simulink model "simscape_antenna_240102"  (R2022a)
settings: Solver=VariableStepAuto  StartTime=0.0  StopTime=5  FixedStep=Ts  RelTol=1e-3  AbsTol=1e-3  EnableMultiTasking=on
PreLoadFcn:
  | % Control parameters
  | Ts = 2e-6;   % Fundamental sample time
  | fsw = 2e3;   % Switching frequency (Hz)
  | fc = fsw*10; % Control loop frequency (Hz)
  | Tsc = 1/fc;  % Control loop sample time
  | 
  | % PMSM parameters
  | PM = 0.03; % Permanent magnet flux linkage
  | Ld = 2e-4;  % d-axis inductance
  | Lq = 2e-4;  % q-axis inductance
  | L0 = 2e-4;  % 0-axis inductance
  | Rs = 0.013; % Stator resistance
  | N = 6; % Number of pole pairs
  | J = 0.2; % Moment of inertia
  | 
  | % Operating and derived limits
  | Imax = 100;  % Max stator current (peak value)
  | Tmax = 1.5*N*PM*Imax; % Max lectromagnetic torque
  | fnom = 100;  % Nominal frequency (Hz)
  | rpm_nom = 60*fnom/N;      % Nominal rotor speed (rpm)
  | omegam_nom = 2*pi*fnom/N; % Nominal mechanical rotor speed
  | Pmax = omegam_nom*Tmax;     % Maximum power
StopFcn:
  | ee_addSimlogTimeStamp(bdroot)
undefined symbols (not defined in the file or in its folder): smiData, X, Y, Z
libraries: nesl_utility x21, ee_lib x20, fl_lib x20, sm_lib x15, slpidlib x6, eePwmGeneratorTwoLevel x2, spsabctodq0Lib x2, eeTransforms x2, spsdq0toabcLib x1, eePmsmCurrentController x1, eePmsmCurrentReferenceGen x1, eePmsmFieldOrientedControl x1
(part 2 of 3)

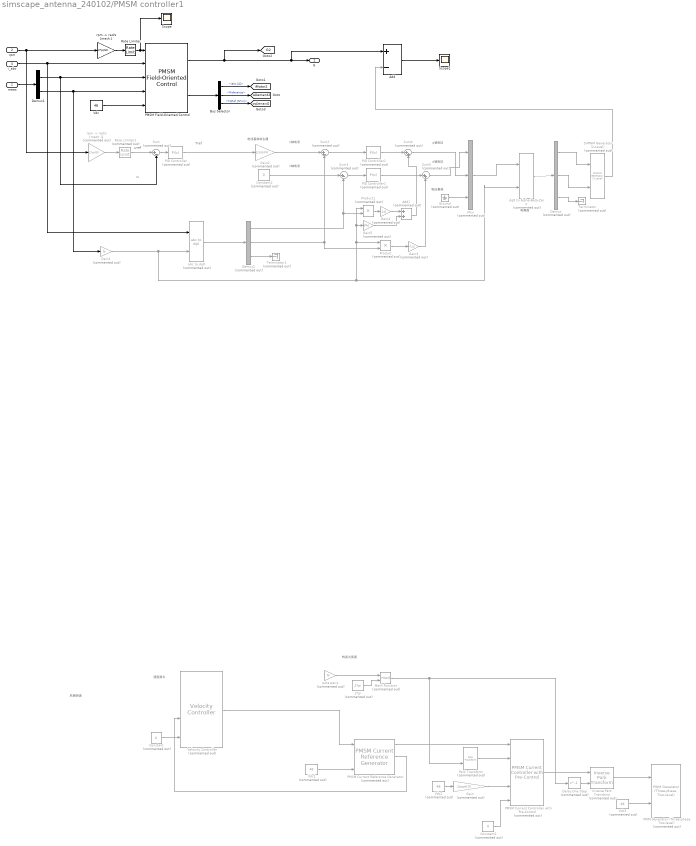
== system simscape_antenna_240102/PMSM controller1 ==
  note: 电角度
  note: 电压基准
  note: q轴电压
  note: 电流基准发生器
  note: Tref
  note: ω
  note: d轴电流
  note: q轴电流
  note: ωref
  note: 转变为弧度
  note: 速度指令
  note: 机械转速
  note: d轴电压
  meas : Inport
  rpm : Inport  Port=2
  i_abc : Inport  Port=3
  2*pi : Constant  Commented=on  Value=2*pi  SampleTime=-1
  Add : Sum  Inputs=+-
  Add1 : Sum  Commented=on
  Bus Selector : BusSelector  OutputSignals=iabc [A],Reference,TqRef [N*m]
  Constant : Constant  Commented=on  Value=0
  Constant1 : Constant  Commented=on  Value=0
  Constant2 : Constant  Commented=on  Value=0
  Delay One Step : Delay  Commented=on  DelayLength=1
  Demux : Demux  Commented=on  Outputs=3
  Demux1 : Demux  Outputs=2
  Demux2 : Demux  Commented=on  Outputs=3
  Gain : Gain  Commented=on  Gain=1/sqrt(3)
  Gain1 : Gain  Commented=on  Gain=N
  Gain2 : Gain  Commented=on  Gain=2/3/N/PM
  Gain3 : Gain  Commented=on  Gain=-Lq
  Gain4 : Gain  Commented=on  Gain=Ld
  Gain5 : Gain  Commented=on  Gain=PM
  Ground : Ground  Commented=on
  Inverse Park Transform : eeTransforms/Inverse Park Transform  Commented=on  AxisAlignment=Q-axis  PowerInvariant=off
  Math Function : Math  Commented=on  Operator=mod  SignedPower=on
  Mux : Mux  Commented=on  Inputs=3
  PID Controller : slpidlib/PID Controller  Commented=on  Controller=PI  Form=Parallel  TimeDomain=Discrete-time  UseExternalTs=off  SampleTime=-1  IntegratorMethod=Forward Euler  FilterMethod=Forward Euler  ControllerParametersSource=internal  P=60  I=6000  UseKiTs=off  D=0  N=100  UseFilter=on  TunerSelectOption=Transfer Function Based (PID Tuner App)  InitialConditionSource=internal  InitialConditionForIntegrator=0  InitialConditionForFilter=0  DifferentiatorICPrevScaledInput=0  ExternalReset=none  TrackingMode=off  Kt=1  LimitOutput=off  SatLimitsSource=internal  UpperSaturationLimit=inf  LowerSaturationLimit=-inf  LinearizeAsGain=on  AntiWindupMode=none  Kb=1  POutMin=[]  POutMax=[]  IOutMin=[]  IOutMax=[]  DOutMin=[]  DOutMax=[]  NOutMin=[]  NOutMax=[]  SumOutMin=[]  SumOutMax=[]  SaturationOutMin=[]  SaturationOutMax=[]  PParamMin=[]  PParamMax=[]  IParamMin=[]  IParamMax=[]  DParamMin=[]  DParamMax=[]  NParamMin=[]  NParamMax=[]  KbParamMin=[]  KbParamMax=[]  KtParamMin=[]  KtParamMax=[]  KbOutMin=[]  KbOutMax=[]  KtOutMin=[]  KtOutMax=[]  IntegratorOutMin=[]  IntegratorOutMax=[]  FilterOutMin=[]  FilterOutMax=[]  SumI1OutMin=[]  SumI1OutMax=[]  SumI2OutMin=[]  SumI2OutMax=[]  SumI3OutMin=[]  SumI3OutMax=[]  SumI4OutMin=[]  SumI4OutMax=[]  SumDOutMin=[]  SumDOutMax=[]  DifferentiatorOutMin=[]  DifferentiatorOutMax=[]  FilterDiffOutCoefMin=[]  FilterDiffOutCoefMax=[]  ReciprocalOutMin=[]  ReciprocalOutMax=[]  SumDenOutMin=[]  SumDenOutMax=[]  SumNumOutMin=[]  SumNumOutMax=[]  DivideOutMin=[]  DivideOutMax=[]  UdiffTsProdOutMin=[]  UdiffTsProdOutMax=[]  NTsProdOutMin=[]  NTsProdOutMax=[]  UintegralTsProdOutMin=[]  UintegralTsProdOutMax=[]  UngainTsProdOutMin=[]  UngainTsProdOutMax=[]  IntegratorContinuousStateAttributes=''  IntegratorStateMustResolveToSignalObject=off  IntegratorRTWStateStorageClass=Auto  FilterContinuousStateAttributes=''  FilterStateMustResolveToSignalObject=off  FilterRTWStateStorageClass=Auto  ParallelPVariant=InternalParameters  IdealPVariant=Disabled  IVariant=InternalParameters  DVariant=Disabled  IntegratorVariant=Discrete  SatVariant=Disabled  AWVariant=Passthrough  PCopyVariant=Disabled  TRVariant=Disabled  FdbkBlocksVariant=Forward  IdealPFdbkVariant=Disabled  SatFdbkVariant=Disabled  DerivativeFilterVariant=Disabled  NVariant=Disabled  NCopyVariant=Disabled_SignalSpec  FilterICVariant=Disabled  IntegratorICVariant=InternalICs  ExternalResetVariant=Disabled  TRSumVariant=Passthrough  SumFdbkVariant=Disabled  SumVariant=Sum_PI  TsampFilterVariant=InternalTs  TsampNgainVariant=Passthrough  TsampIntegralVariant=Passthrough  ExternalSaturationOutDataTypeStr=Inherit: Same as second input  aMode=0
  PID Controller1 : slpidlib/PID Controller  Commented=on  Controller=PI  Form=Parallel  TimeDomain=Discrete-time  UseExternalTs=off  SampleTime=-1  IntegratorMethod=Forward Euler  FilterMethod=Forward Euler  ControllerParametersSource=internal  P=0.1  I=10  UseKiTs=off  D=0  N=100  UseFilter=on  TunerSelectOption=Transfer Function Based (PID Tuner App)  InitialConditionSource=internal  InitialConditionForIntegrator=0  InitialConditionForFilter=0  DifferentiatorICPrevScaledInput=0  ExternalReset=none  TrackingMode=off  Kt=1  LimitOutput=off  SatLimitsSource=internal  UpperSaturationLimit=inf  LowerSaturationLimit=-inf  LinearizeAsGain=on  AntiWindupMode=none  Kb=1  POutMin=[]  POutMax=[]  IOutMin=[]  IOutMax=[]  DOutMin=[]  DOutMax=[]  NOutMin=[]  NOutMax=[]  SumOutMin=[]  SumOutMax=[]  SaturationOutMin=[]  SaturationOutMax=[]  PParamMin=[]  PParamMax=[]  IParamMin=[]  IParamMax=[]  DParamMin=[]  DParamMax=[]  NParamMin=[]  NParamMax=[]  KbParamMin=[]  KbParamMax=[]  KtParamMin=[]  KtParamMax=[]  KbOutMin=[]  KbOutMax=[]  KtOutMin=[]  KtOutMax=[]  IntegratorOutMin=[]  IntegratorOutMax=[]  FilterOutMin=[]  FilterOutMax=[]  SumI1OutMin=[]  SumI1OutMax=[]  SumI2OutMin=[]  SumI2OutMax=[]  SumI3OutMin=[]  SumI3OutMax=[]  SumI4OutMin=[]  SumI4OutMax=[]  SumDOutMin=[]  SumDOutMax=[]  DifferentiatorOutMin=[]  DifferentiatorOutMax=[]  FilterDiffOutCoefMin=[]  FilterDiffOutCoefMax=[]  ReciprocalOutMin=[]  ReciprocalOutMax=[]  SumDenOutMin=[]  SumDenOutMax=[]  SumNumOutMin=[]  SumNumOutMax=[]  DivideOutMin=[]  DivideOutMax=[]  UdiffTsProdOutMin=[]  UdiffTsProdOutMax=[]  NTsProdOutMin=[]  NTsProdOutMax=[]  UintegralTsProdOutMin=[]  UintegralTsProdOutMax=[]  UngainTsProdOutMin=[]  UngainTsProdOutMax=[]  IntegratorContinuousStateAttributes=''  IntegratorStateMustResolveToSignalObject=off  IntegratorRTWStateStorageClass=Auto  FilterContinuousStateAttributes=''  FilterStateMustResolveToSignalObject=off  FilterRTWStateStorageClass=Auto  ParallelPVariant=InternalParameters  IdealPVariant=Disabled  IVariant=InternalParameters  DVariant=Disabled  IntegratorVariant=Discrete  SatVariant=Disabled  AWVariant=Passthrough  PCopyVariant=Disabled  TRVariant=Disabled  FdbkBlocksVariant=Forward  IdealPFdbkVariant=Disabled  SatFdbkVariant=Disabled  DerivativeFilterVariant=Disabled  NVariant=Disabled  NCopyVariant=Disabled_SignalSpec  FilterICVariant=Disabled  IntegratorICVariant=InternalICs  ExternalResetVariant=Disabled  TRSumVariant=Passthrough  SumFdbkVariant=Disabled  SumVariant=Sum_PI  TsampFilterVariant=InternalTs  TsampNgainVariant=Passthrough  TsampIntegralVariant=Passthrough  ExternalSaturationOutDataTypeStr=Inherit: Same as second input  aMode=0
  PID Controller2 : slpidlib/PID Controller  Commented=on  Controller=PI  Form=Parallel  TimeDomain=Discrete-time  UseExternalTs=off  SampleTime=-1  IntegratorMethod=Forward Euler  FilterMethod=Forward Euler  ControllerParametersSource=internal  P=0.1  I=10  UseKiTs=off  D=0  N=100  UseFilter=on  TunerSelectOption=Transfer Function Based (PID Tuner App)  InitialConditionSource=internal  InitialConditionForIntegrator=0  InitialConditionForFilter=0  DifferentiatorICPrevScaledInput=0  ExternalReset=none  TrackingMode=off  Kt=1  LimitOutput=off  SatLimitsSource=internal  UpperSaturationLimit=inf  LowerSaturationLimit=-inf  LinearizeAsGain=on  AntiWindupMode=none  Kb=1  POutMin=[]  POutMax=[]  IOutMin=[]  IOutMax=[]  DOutMin=[]  DOutMax=[]  NOutMin=[]  NOutMax=[]  SumOutMin=[]  SumOutMax=[]  SaturationOutMin=[]  SaturationOutMax=[]  PParamMin=[]  PParamMax=[]  IParamMin=[]  IParamMax=[]  DParamMin=[]  DParamMax=[]  NParamMin=[]  NParamMax=[]  KbParamMin=[]  KbParamMax=[]  KtParamMin=[]  KtParamMax=[]  KbOutMin=[]  KbOutMax=[]  KtOutMin=[]  KtOutMax=[]  IntegratorOutMin=[]  IntegratorOutMax=[]  FilterOutMin=[]  FilterOutMax=[]  SumI1OutMin=[]  SumI1OutMax=[]  SumI2OutMin=[]  SumI2OutMax=[]  SumI3OutMin=[]  SumI3OutMax=[]  SumI4OutMin=[]  SumI4OutMax=[]  SumDOutMin=[]  SumDOutMax=[]  DifferentiatorOutMin=[]  DifferentiatorOutMax=[]  FilterDiffOutCoefMin=[]  FilterDiffOutCoefMax=[]  ReciprocalOutMin=[]  ReciprocalOutMax=[]  SumDenOutMin=[]  SumDenOutMax=[]  SumNumOutMin=[]  SumNumOutMax=[]  DivideOutMin=[]  DivideOutMax=[]  UdiffTsProdOutMin=[]  UdiffTsProdOutMax=[]  NTsProdOutMin=[]  NTsProdOutMax=[]  UintegralTsProdOutMin=[]  UintegralTsProdOutMax=[]  UngainTsProdOutMin=[]  UngainTsProdOutMax=[]  IntegratorContinuousStateAttributes=''  IntegratorStateMustResolveToSignalObject=off  IntegratorRTWStateStorageClass=Auto  FilterContinuousStateAttributes=''  FilterStateMustResolveToSignalObject=off  FilterRTWStateStorageClass=Auto  ParallelPVariant=InternalParameters  IdealPVariant=Disabled  IVariant=InternalParameters  DVariant=Disabled  IntegratorVariant=Discrete  SatVariant=Disabled  AWVariant=Passthrough  PCopyVariant=Disabled  TRVariant=Disabled  FdbkBlocksVariant=Forward  IdealPFdbkVariant=Disabled  SatFdbkVariant=Disabled  DerivativeFilterVariant=Disabled  NVariant=Disabled  NCopyVariant=Disabled_SignalSpec  FilterICVariant=Disabled  IntegratorICVariant=InternalICs  ExternalResetVariant=Disabled  TRSumVariant=Passthrough  SumFdbkVariant=Disabled  SumVariant=Sum_PI  TsampFilterVariant=InternalTs  TsampNgainVariant=Passthrough  TsampIntegralVariant=Passthrough  ExternalSaturationOutDataTypeStr=Inherit: Same as second input  aMode=0
  PMSM Current Controller with Pre-Control : eePmsmCurrentController/PMSM Current Controller with Pre-Control  Commented=on  Kp_id=0.1  Ki_id=10  Kaw_id=1000  Kp_iq=0.1  Ki_iq=10  Kaw_iq=1000  Ts=-1  Tsd=0.001  AxisPrio=Q-axis  ActZC=off  ActFF=on  idVect=[-200, 0, 200]  iqVect=[-200, 0, 200]  LdMatrix=0.0002 * ones(3, 3)  LqMatrix=0.0002 * ones(3, 3)  psimMatrix=0.04 * ones(3, 3)
      settings: SourceProductBaseCode=PS
  PMSM Current Reference Generator : eePmsmCurrentReferenceGen/PMSM Current Reference Generator  Commented=on  Vnom=10  Pmax=Pmax  Tmax=Tmax*1.5  Ts=2e-6  RefType=Zero d-axis control  rpmVec=[0, 3000]  TqVec=[-100, 0, 100]  VdcVec=[300, 350]  PWMMode=SVM: space vector modulation  ModFactor=1  idMatrix=zeros(2,3,2)  iqMatrix=zeros(2,3,2)  p=8  psim=0.04  Ld=0.00024  Lq=0.00029  Rs=0.01  RefExpEnable=0
      settings: SourceProductBaseCode=PS
  PMSM Field-Oriented Control : eePmsmFieldOrientedControl/PMSM Field-Oriented Control  winding_type=Wye-wound  CtrlMode=Velocity control  Vnom=48  Pmax=Pmax  Tmax=Tmax*1.5  p=N  Vdc_on=10  Ts=Ts  Tsc=Tsc  CtrlType=PI control  Kp_w=60  Ki_w=300*2  Kv_w=1  Kaw_w=1000  RefType=Zero d-axis control  rpmVec=[0, 3000]  TqVec=[-100, 0, 100]  VdcVec=[300, 350]  PWMMode=SPWM: sinusoidal PWM  ModFactor=1  idMatrix=zeros(2,3,2)  iqMatrix=zeros(2,3,2)  psim=PM  Ld=0.00024  Lq=0.00029  Rs=0.01  AxisAlignment=Q-axis  Kp_id=0.1  Ki_id=10  Kaw_id=1000  Kp_iq=0.1  Ki_iq=10  Kaw_iq=1000  AxisPrio=Q-axis  ActZC=off  ActFF=on  ParamTypeFF=Constant parameters  LdFF=Ld  LqFF=Lq  psimFF=PM  idVect=[-200, 0, 200]  iqVect=[-200, 0, 200]  LdMatrix=0.0002 * ones(3, 3)  LqMatrix=0.0002 * ones(3, 3)  psimMatrix=0.04 * ones(3, 3)  CPWMMode=SPWM: sinusoidal PWM  fsw=fsw
      settings: SourceProductBaseCode=PS
  "PWM Generator (Three-phase, Two-level)" : eePwmGeneratorTwoLevel/PWM Generator (Three-phase, Two-level)  Commented=on  PWMMode=Continuous PWM (CPWM)  CPWMMode=SPWM: sinusoidal PWM  DPWMMode=60 DPWM: 60 degree discontinuous PWM  fsw=1e3  Ts=2e-6
      settings: SourceProductBaseCode=PS
  Park Transform : eeTransforms/Park Transform  Commented=on  AxisAlignment=Q-axis  PowerInvariant=off
  Product : Product  Commented=on
  Product1 : Product  Commented=on
  Rate Limiter : RateLimiter  RisingSlewLimit=Tmax/J  FallingSlewLimit=-Tmax/J  SampleTimeMode=inherited
  Rate Limiter1 : RateLimiter  Commented=on  RisingSlewLimit=Tmax/J  FallingSlewLimit=-Tmax/J  SampleTimeMode=inherited
  SVPWM Generator (2-Level) : spsSVPWMGenerator2LevelLib/SVPWM Generator (2-Level)  Commented=on  InputType=alpha-beta components  SwitchingPattern=Pattern #1  Fc=2000  ParUref=[0.8 -30 50]  Ts=0
      settings: SourceProductBaseCode=PS
  Scope : Scope
  Scope1 : Scope
  Sum : Sum  Commented=on  Inputs=|+-
  Sum2 : Sum  Commented=on  Inputs=|+-
  Sum3 : Sum  Commented=on  Inputs=|+-
  Sum4 : Sum  Commented=on  Inputs=|++
  Sum5 : Sum  Commented=on  Inputs=|++
  Terminator : Terminator  Commented=on
  Terminator1 : Terminator  Commented=on
  Vdc : Constant  Value=48  SampleTime=Tsc
  Vdc1 : Constant  Commented=on  Value=48  SampleTime=Tsc
  Vdc2 : Constant  Commented=on  Value=48  SampleTime=Tsc
  Vdc3 : Constant  Commented=on  Value=48  SampleTime=Tsc
  Velocity Controller : eeVelocityController/Velocity Controller  Commented=on  CtrlType=PI control  Kp_w=60  Ki_w=300*2  Kv_w=1  Kaw_w=1000  Ts=2e-6  Tsd=0.001  ActZC=off
      settings: SourceProductBaseCode=PS
  abc to dq0 : spsabctodq0Lib/abc to dq0  Commented=on  Alignment=90 degrees behind phase A axis
  dq0 to Alpha-Beta-Zero : spsdq0toAlphaBetaZeroLib/dq0 to Alpha-Beta-Zero  Commented=on  Alignment=90 degrees behind phase A axis
      settings: SourceProductBaseCode=PS
  "pole pairs " : Gain  Commented=on  Gain=N
  "rpm -> rad/s [mech.]" : Gain  Gain=2*pi/60
  "rpm -> rad/s [mech.]1" : Gain  Commented=on  Gain=2*pi/60
  G : Outport  VectorParamsAs1DForOutWhenUnconnected=off
  tag scope: G2=global, iMotor2=global, trqDemand2=global, wDemand2=global
  wires:
  "rpm -> rad/s [mech.]"/1 -> Rate Limiter/1
  Rate Limiter/1 -> Scope/1, PMSM Field-Oriented Control/1
  rpm/1 -> "rpm -> rad/s [mech.]1"/1, "rpm -> rad/s [mech.]"/1
  Bus Selector/3 -> [trqDemand2]  "<TqRef [N*m]>"
  Bus Selector/2 -> [wDemand2]  "<Reference>"
  Bus Selector/1 -> [iMotor2]  "<iabc [A]>"
  meas/1 -> Demux1/1
  i_abc/1 -> abc to dq0/1, PMSM Field-Oriented Control/2
  PMSM Field-Oriented Control/2 -> Bus Selector/1
  Vdc/1 -> PMSM Field-Oriented Control/5
  PMSM Field-Oriented Control/1 -> G/1, Add/1, [G2]
  "rpm -> rad/s [mech.]1"/1 -> Rate Limiter1/1
  Rate Limiter1/1 -> Sum/1
  Sum/1 -> PID Controller/1
  Velocity Controller/1 -> PMSM Current Reference Generator/1
  PMSM Current Reference Generator/1 -> PMSM Current Controller with Pre-Control/1
  PMSM Current Controller with Pre-Control/1 -> Inverse Park Transform/1
  Inverse Park Transform/1 -> "PWM Generator (Three-phase, Two-level)"/1
  Constant/1 -> Velocity Controller/4
  PMSM Current Reference Generator/2 -> Velocity Controller/3
  Vdc1/1 -> PMSM Current Reference Generator/3
  Park Transform/1 -> PMSM Current Controller with Pre-Control/2
  Vdc2/1 -> Gain/1
  Gain/1 -> PMSM Current Controller with Pre-Control/4
  Constant1/1 -> PMSM Current Controller with Pre-Control/5
  Vdc3/1 -> "PWM Generator (Three-phase, Two-level)"/2
  2*pi/1 -> Math Function/2
  "pole pairs "/1 -> Math Function/1
  Demux1/2 -> Gain1/1, PMSM Field-Oriented Control/4
  Math Function/1 -> Delay One Step/1, Park Transform/2
  Add/1 -> Scope1/1
  Delay One Step/1 -> Inverse Park Transform/2
  Demux1/1 -> PMSM Field-Oriented Control/3, Sum/2
  PID Controller/1 -> Gain2/1
  Gain2/1 -> Sum2/1
  Sum2/1 -> PID Controller1/1
  Constant2/1 -> Sum3/1
  Demux2/2 -> Product/2, Sum2/2
  Demux2/1 -> Product1/2, Sum3/2
  Sum3/1 -> PID Controller2/1
  PID Controller1/1 -> Sum4/1
  PID Controller2/1 -> Sum5/1
  Sum4/1 -> Mux/2
  Sum5/1 -> Mux/1
  Ground/1 -> Mux/3
  Mux/1 -> dq0 to Alpha-Beta-Zero/1
  dq0 to Alpha-Beta-Zero/1 -> Demux/1
  Demux/1 -> SVPWM Generator (2-Level)/1
  Demux/2 -> SVPWM Generator (2-Level)/2
  Demux/3 -> Terminator/1
  SVPWM Generator (2-Level)/1 -> Add/2
  abc to dq0/1 -> Demux2/1
  Demux2/3 -> Terminator1/1
  Gain1/1 -> Gain5/1, Product1/1, Product/1, dq0 to Alpha-Beta-Zero/2, abc to dq0/2
  Gain3/1 -> Sum5/2
  Product/1 -> Gain3/1
  Product1/1 -> Gain4/1
  Gain4/1 -> Add1/1
  Gain5/1 -> Add1/2
  Add1/1 -> Sum4/2

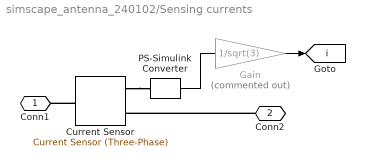
== system simscape_antenna_240102/Sensing currents ==
  Current Sensor : ee_lib/Sensors & Transducers/Current Sensor (Three-Phase)
  Gain : Gain  Commented=on  Gain=1/sqrt(3)
  PS-Simulink Converter : nesl_utility/PS-Simulink Converter  PhysicalDomain=network_engine_domain  SubClassName=ps_output  LeftPortType=input  RightPortType=output  PseudoPeriodic=off  Frequencies=[]  VectorFormat=1-D array  Unit=A  AffineConversion=off
      settings: SourceProductBaseCode=SS,PW,VE
  Conn1 : PMIOPort  Side=Left
  Conn2 : PMIOPort  Port=2  Side=Right
  tag scope: i=global
  wires:
  PS-Simulink Converter/1 -> [i]
  connections:
  Current Sensor/RConn1 -- PS-Simulink Converter/LConn1
  Conn2/RConn1 -- Current Sensor/RConn2
  Current Sensor/LConn1 -- Conn1/RConn1

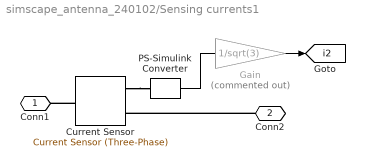
== system simscape_antenna_240102/Sensing currents1 ==
  Current Sensor : ee_lib/Sensors & Transducers/Current Sensor (Three-Phase)
  Gain : Gain  Commented=on  Gain=1/sqrt(3)
  PS-Simulink Converter : nesl_utility/PS-Simulink Converter  PhysicalDomain=network_engine_domain  SubClassName=ps_output  LeftPortType=input  RightPortType=output  PseudoPeriodic=off  Frequencies=[]  VectorFormat=1-D array  Unit=A  AffineConversion=off
      settings: SourceProductBaseCode=SS,PW,VE
  Conn1 : PMIOPort  Side=Left
  Conn2 : PMIOPort  Port=2  Side=Right
  tag scope: i2=global
  wires:
  PS-Simulink Converter/1 -> [i2]
  connections:
  Current Sensor/LConn1 -- Conn1/RConn1
  Conn2/RConn1 -- Current Sensor/RConn2
  Current Sensor/RConn1 -- PS-Simulink Converter/LConn1

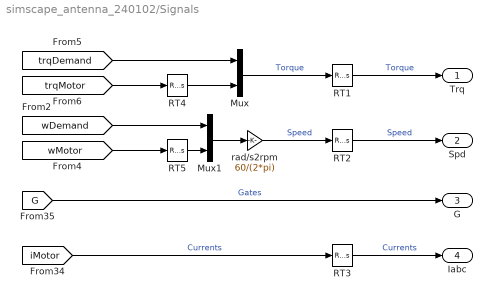
== system simscape_antenna_240102/Signals  ==
  Mux : Mux  Inputs=2
  Mux1 : Mux  Inputs=2
  RT1 : RateTransition  OutPortSampleTime=Ts
  RT2 : RateTransition  OutPortSampleTime=Ts
  RT3 : RateTransition  OutPortSampleTime=Ts
  RT4 : RateTransition  OutPortSampleTime=Tsc
  RT5 : RateTransition  OutPortSampleTime=Tsc
  rad/s2rpm : Gain  Gain=60/(2*pi)
  Trq : Outport  VectorParamsAs1DForOutWhenUnconnected=off
  Spd : Outport  Port=2  VectorParamsAs1DForOutWhenUnconnected=off
  G : Outport  Port=3  VectorParamsAs1DForOutWhenUnconnected=off
  Iabc : Outport  Port=4  VectorParamsAs1DForOutWhenUnconnected=off
  wires:
  [trqDemand] -> Mux/1
  [G] -> G/1  "Gates"
  Mux1/1 -> rad/s2rpm/1
  Mux/1 -> RT1/1  "Torque"
  [iMotor] -> RT3/1  "Currents"
  [wDemand] -> Mux1/1
  rad/s2rpm/1 -> RT2/1  "Speed"
  [trqMotor] -> RT4/1
  [wMotor] -> RT5/1
  RT1/1 -> Trq/1  "Torque"
  RT2/1 -> Spd/1  "Speed"
  RT3/1 -> Iabc/1  "Currents"
  RT4/1 -> Mux/2
  RT5/1 -> Mux1/2

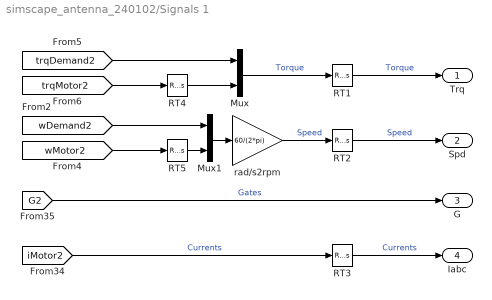
== system simscape_antenna_240102/Signals 1 ==
  Mux : Mux  Inputs=2
  Mux1 : Mux  Inputs=2
  RT1 : RateTransition  OutPortSampleTime=Ts
  RT2 : RateTransition  OutPortSampleTime=Ts
  RT3 : RateTransition  OutPortSampleTime=Ts
  RT4 : RateTransition  OutPortSampleTime=Tsc
  RT5 : RateTransition  OutPortSampleTime=Tsc
  rad/s2rpm : Gain  Gain=60/(2*pi)
  Trq : Outport  VectorParamsAs1DForOutWhenUnconnected=off
  Spd : Outport  Port=2  VectorParamsAs1DForOutWhenUnconnected=off
  G : Outport  Port=3  VectorParamsAs1DForOutWhenUnconnected=off
  Iabc : Outport  Port=4  VectorParamsAs1DForOutWhenUnconnected=off
  wires:
  RT5/1 -> Mux1/2
  RT4/1 -> Mux/2
  RT3/1 -> Iabc/1  "Currents"
  RT2/1 -> Spd/1  "Speed"
  RT1/1 -> Trq/1  "Torque"
  [wMotor2] -> RT5/1
  [trqMotor2] -> RT4/1
  rad/s2rpm/1 -> RT2/1  "Speed"
  [wDemand2] -> Mux1/1
  [iMotor2] -> RT3/1  "Currents"
  Mux/1 -> RT1/1  "Torque"
  Mux1/1 -> rad/s2rpm/1
  [G2] -> G/1  "Gates"
  [trqDemand2] -> Mux/1

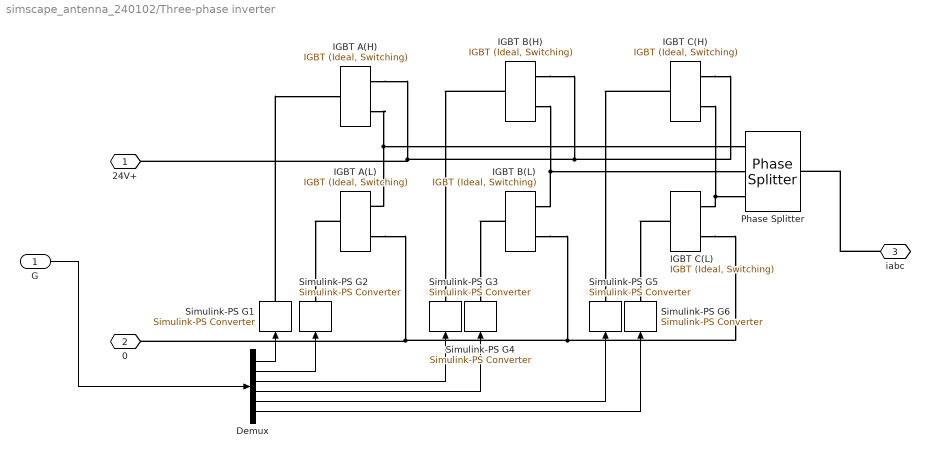
== system simscape_antenna_240102/Three-phase inverter ==
  G : Inport
  Demux : Demux  Outputs=6
  IGBT A(H) : ee_lib/Semiconductors & Converters/IGBT (Ideal, Switching)  Vf=0.8 V  Ron=0.001 Ohm  Goff=1e-5 S  Vth=0.5 V  diode_param=2  diode_Vf=0.8 V  diode_Ron=0.001 Ohm  diode_Goff=1e-5 S  diode_C=5e-8 F  diode_iRM=-235 A  diode_iF=300 A  diode_idot=-50 A/us  diode_trr_param=1  diode_trr_factor=3  diode_trr=15 us  diode_Qrr=1.5e+3 s*uA  thermal_loss_option=ee.enum.converters.thermalLossOption.constantvalues  Von_data=[0, .1, .6, .8, 1, 1.3, 1.6, 2, 2.4; 0, .1, .7, 1, 1.2, 1.5, 1.9, 2.4, 2.8] V  Tj=[298.15, 398.15] K  Iout_data=[0, .1, 1, 5, 10, 20, 40, 70, 100] A  Eon_data=[0, .0024, .024, .12, .2, .48, 1.04, 2.16, 3.24; 0, .003, .03, .15, .25, .6, 1.3, 2.7, 4.05] * 1e-3 J  Eoff_data=[0, .0007, .0066, .033, .066, .17, .33, .83, 1.5; 0, .001, .01, .05, .1, .25, .5, 1.2, 2.2] * 1e-3 J  Tj_loss=[298.15, 398.15] K  Iout_data_loss=[0, .1, 1, 5, 10, 20, 40, 70, 100] A  Eon_scalar=22.86e-3 J  Eoff_scalar=17.14e-3 J  Voff=300 V  Iout_scalar=600 A  diodeModelType=ee.enum.converters.diodeModelType.pwl  diodeTableType=ee.enum.diode.tableType.IfMat  diode_IfMat=[.07, .12, .19, 1.75, 4.24, 7.32, 11.2; .16, .3, .72, 2.14, 4.02, 6.35, 9.12] A  diode_VfMat=[.9, 1.15, 1.25, 1.5, 1.75, 2.17, 2.6, 2.85; .58, .68, .75, 1.1, 1.38, 1.77, 2.27, 2.7] V  diode_TjVec=[25, 125] degC  diode_VfVec=[.5, .7, .9, 1.3, 1.7, 2.1, 2.5] V  diode_IfVec=[.1, .2, .5, 1, 2, 4, 7, 10] A  diode_Vr=-600 V  diode_Ls=150 nH  diode_Erec=0.03 J  thermal_network_parameterization=ee.enum.thermalNetworkTopology.external  Rth=[.08, .5] K/W  Rth_Cauer=[.08, .1, .5] K/W  Rth_Foster=[.08, .14, .22, .16] K/W  thermal_mass_parameterization=ee.enum.thermalNetwork.timeconstant  thermal_mass=[.01, .5] J/K  thermal_mass_Cauer=[.01, .1, .5] J/K  thermal_mass_Foster=[.001, .005, .05, .5] J/K  thermal_time_constant=[.001, .2] s  thermal_time_constant_Cauer=[.001, .1, .2] s  thermal_time_constant_Foster=[7e-05, .0007, .01, .08] s  thermal_mass_initial_temperatures=[25, 25] degC  thermal_mass_initial_temperatures_Cauer=[25, 25, 25] degC  junction_thermal_mass=0.01 J/K  steadyState_Foster=simscape.enum.onoff.on  Tvec_initial_Foster=[25, 25, 25, 25] degC  no_thermal_network=0  junction_temperature_specify=off  junction_temperature_priority=None  junction_temperature=25 degC  junction_temperature_nominal_specify=off  junction_temperature_nominal_unit=degC  junction_temperature_nominal_value=1  vT_specify=off  vT_priority=None  vT=0 V  vT_nominal_specify=off  vT_nominal_unit=V  vT_nominal_value=1  Qj_specify=off  Qj_priority=None  Qj=0 W  Qj_nominal_specify=off  Qj_nominal_unit=W  Qj_nominal_value=1
  IGBT A(L) : ee_lib/Semiconductors & Converters/IGBT (Ideal, Switching)  Vf=0.8 V  Ron=0.001 Ohm  Goff=1e-5 S  Vth=0.5 V  diode_param=2  diode_Vf=0.8 V  diode_Ron=0.001 Ohm  diode_Goff=1e-5 S  diode_C=5e-8 F  diode_iRM=-235 A  diode_iF=300 A  diode_idot=-50 A/us  diode_trr_param=1  diode_trr_factor=3  diode_trr=15 us  diode_Qrr=1.5e+3 s*uA  thermal_loss_option=ee.enum.converters.thermalLossOption.constantvalues  Von_data=[0, .1, .6, .8, 1, 1.3, 1.6, 2, 2.4; 0, .1, .7, 1, 1.2, 1.5, 1.9, 2.4, 2.8] V  Tj=[298.15, 398.15] K  Iout_data=[0, .1, 1, 5, 10, 20, 40, 70, 100] A  Eon_data=[0, .0024, .024, .12, .2, .48, 1.04, 2.16, 3.24; 0, .003, .03, .15, .25, .6, 1.3, 2.7, 4.05] * 1e-3 J  Eoff_data=[0, .0007, .0066, .033, .066, .17, .33, .83, 1.5; 0, .001, .01, .05, .1, .25, .5, 1.2, 2.2] * 1e-3 J  Tj_loss=[298.15, 398.15] K  Iout_data_loss=[0, .1, 1, 5, 10, 20, 40, 70, 100] A  Eon_scalar=22.86e-3 J  Eoff_scalar=17.14e-3 J  Voff=300 V  Iout_scalar=600 A  diodeModelType=ee.enum.converters.diodeModelType.pwl  diodeTableType=ee.enum.diode.tableType.IfMat  diode_IfMat=[.07, .12, .19, 1.75, 4.24, 7.32, 11.2; .16, .3, .72, 2.14, 4.02, 6.35, 9.12] A  diode_VfMat=[.9, 1.15, 1.25, 1.5, 1.75, 2.17, 2.6, 2.85; .58, .68, .75, 1.1, 1.38, 1.77, 2.27, 2.7] V  diode_TjVec=[25, 125] degC  diode_VfVec=[.5, .7, .9, 1.3, 1.7, 2.1, 2.5] V  diode_IfVec=[.1, .2, .5, 1, 2, 4, 7, 10] A  diode_Vr=-600 V  diode_Ls=150 nH  diode_Erec=0.03 J  thermal_network_parameterization=ee.enum.thermalNetworkTopology.external  Rth=[.08, .5] K/W  Rth_Cauer=[.08, .1, .5] K/W  Rth_Foster=[.08, .14, .22, .16] K/W  thermal_mass_parameterization=ee.enum.thermalNetwork.timeconstant  thermal_mass=[.01, .5] J/K  thermal_mass_Cauer=[.01, .1, .5] J/K  thermal_mass_Foster=[.001, .005, .05, .5] J/K  thermal_time_constant=[.001, .2] s  thermal_time_constant_Cauer=[.001, .1, .2] s  thermal_time_constant_Foster=[7e-05, .0007, .01, .08] s  thermal_mass_initial_temperatures=[25, 25] degC  thermal_mass_initial_temperatures_Cauer=[25, 25, 25] degC  junction_thermal_mass=0.01 J/K  steadyState_Foster=simscape.enum.onoff.on  Tvec_initial_Foster=[25, 25, 25, 25] degC  no_thermal_network=0  junction_temperature_specify=off  junction_temperature_priority=None  junction_temperature=25 degC  junction_temperature_nominal_specify=off  junction_temperature_nominal_unit=degC  junction_temperature_nominal_value=1  vT_specify=off  vT_priority=None  vT=0 V  vT_nominal_specify=off  vT_nominal_unit=V  vT_nominal_value=1  Qj_specify=off  Qj_priority=None  Qj=0 W  Qj_nominal_specify=off  Qj_nominal_unit=W  Qj_nominal_value=1
  IGBT B(H) : ee_lib/Semiconductors & Converters/IGBT (Ideal, Switching)  Vf=0.8 V  Ron=0.001 Ohm  Goff=1e-5 S  Vth=0.5 V  diode_param=2  diode_Vf=0.8 V  diode_Ron=0.001 Ohm  diode_Goff=1e-5 S  diode_C=5e-8 F  diode_iRM=-235 A  diode_iF=300 A  diode_idot=-50 A/us  diode_trr_param=1  diode_trr_factor=3  diode_trr=15 us  diode_Qrr=1.5e+3 s*uA  thermal_loss_option=ee.enum.converters.thermalLossOption.constantvalues  Von_data=[0, .1, .6, .8, 1, 1.3, 1.6, 2, 2.4; 0, .1, .7, 1, 1.2, 1.5, 1.9, 2.4, 2.8] V  Tj=[298.15, 398.15] K  Iout_data=[0, .1, 1, 5, 10, 20, 40, 70, 100] A  Eon_data=[0, .0024, .024, .12, .2, .48, 1.04, 2.16, 3.24; 0, .003, .03, .15, .25, .6, 1.3, 2.7, 4.05] * 1e-3 J  Eoff_data=[0, .0007, .0066, .033, .066, .17, .33, .83, 1.5; 0, .001, .01, .05, .1, .25, .5, 1.2, 2.2] * 1e-3 J  Tj_loss=[298.15, 398.15] K  Iout_data_loss=[0, .1, 1, 5, 10, 20, 40, 70, 100] A  Eon_scalar=22.86e-3 J  Eoff_scalar=17.14e-3 J  Voff=300 V  Iout_scalar=600 A  diodeModelType=ee.enum.converters.diodeModelType.pwl  diodeTableType=ee.enum.diode.tableType.IfMat  diode_IfMat=[.07, .12, .19, 1.75, 4.24, 7.32, 11.2; .16, .3, .72, 2.14, 4.02, 6.35, 9.12] A  diode_VfMat=[.9, 1.15, 1.25, 1.5, 1.75, 2.17, 2.6, 2.85; .58, .68, .75, 1.1, 1.38, 1.77, 2.27, 2.7] V  diode_TjVec=[25, 125] degC  diode_VfVec=[.5, .7, .9, 1.3, 1.7, 2.1, 2.5] V  diode_IfVec=[.1, .2, .5, 1, 2, 4, 7, 10] A  diode_Vr=-600 V  diode_Ls=150 nH  diode_Erec=0.03 J  thermal_network_parameterization=ee.enum.thermalNetworkTopology.external  Rth=[.08, .5] K/W  Rth_Cauer=[.08, .1, .5] K/W  Rth_Foster=[.08, .14, .22, .16] K/W  thermal_mass_parameterization=ee.enum.thermalNetwork.timeconstant  thermal_mass=[.01, .5] J/K  thermal_mass_Cauer=[.01, .1, .5] J/K  thermal_mass_Foster=[.001, .005, .05, .5] J/K  thermal_time_constant=[.001, .2] s  thermal_time_constant_Cauer=[.001, .1, .2] s  thermal_time_constant_Foster=[7e-05, .0007, .01, .08] s  thermal_mass_initial_temperatures=[25, 25] degC  thermal_mass_initial_temperatures_Cauer=[25, 25, 25] degC  junction_thermal_mass=0.01 J/K  steadyState_Foster=simscape.enum.onoff.on  Tvec_initial_Foster=[25, 25, 25, 25] degC  no_thermal_network=0  junction_temperature_specify=off  junction_temperature_priority=None  junction_temperature=25 degC  junction_temperature_nominal_specify=off  junction_temperature_nominal_unit=degC  junction_temperature_nominal_value=1  vT_specify=off  vT_priority=None  vT=0 V  vT_nominal_specify=off  vT_nominal_unit=V  vT_nominal_value=1  Qj_specify=off  Qj_priority=None  Qj=0 W  Qj_nominal_specify=off  Qj_nominal_unit=W  Qj_nominal_value=1
  IGBT B(L) : ee_lib/Semiconductors & Converters/IGBT (Ideal, Switching)  Vf=0.8 V  Ron=0.001 Ohm  Goff=1e-5 S  Vth=0.5 V  diode_param=2  diode_Vf=0.8 V  diode_Ron=0.001 Ohm  diode_Goff=1e-5 S  diode_C=5e-8 F  diode_iRM=-235 A  diode_iF=300 A  diode_idot=-50 A/us  diode_trr_param=1  diode_trr_factor=3  diode_trr=15 us  diode_Qrr=1.5e+3 s*uA  thermal_loss_option=ee.enum.converters.thermalLossOption.constantvalues  Von_data=[0, .1, .6, .8, 1, 1.3, 1.6, 2, 2.4; 0, .1, .7, 1, 1.2, 1.5, 1.9, 2.4, 2.8] V  Tj=[298.15, 398.15] K  Iout_data=[0, .1, 1, 5, 10, 20, 40, 70, 100] A  Eon_data=[0, .0024, .024, .12, .2, .48, 1.04, 2.16, 3.24; 0, .003, .03, .15, .25, .6, 1.3, 2.7, 4.05] * 1e-3 J  Eoff_data=[0, .0007, .0066, .033, .066, .17, .33, .83, 1.5; 0, .001, .01, .05, .1, .25, .5, 1.2, 2.2] * 1e-3 J  Tj_loss=[298.15, 398.15] K  Iout_data_loss=[0, .1, 1, 5, 10, 20, 40, 70, 100] A  Eon_scalar=22.86e-3 J  Eoff_scalar=17.14e-3 J  Voff=300 V  Iout_scalar=600 A  diodeModelType=ee.enum.converters.diodeModelType.pwl  diodeTableType=ee.enum.diode.tableType.IfMat  diode_IfMat=[.07, .12, .19, 1.75, 4.24, 7.32, 11.2; .16, .3, .72, 2.14, 4.02, 6.35, 9.12] A  diode_VfMat=[.9, 1.15, 1.25, 1.5, 1.75, 2.17, 2.6, 2.85; .58, .68, .75, 1.1, 1.38, 1.77, 2.27, 2.7] V  diode_TjVec=[25, 125] degC  diode_VfVec=[.5, .7, .9, 1.3, 1.7, 2.1, 2.5] V  diode_IfVec=[.1, .2, .5, 1, 2, 4, 7, 10] A  diode_Vr=-600 V  diode_Ls=150 nH  diode_Erec=0.03 J  thermal_network_parameterization=ee.enum.thermalNetworkTopology.external  Rth=[.08, .5] K/W  Rth_Cauer=[.08, .1, .5] K/W  Rth_Foster=[.08, .14, .22, .16] K/W  thermal_mass_parameterization=ee.enum.thermalNetwork.timeconstant  thermal_mass=[.01, .5] J/K  thermal_mass_Cauer=[.01, .1, .5] J/K  thermal_mass_Foster=[.001, .005, .05, .5] J/K  thermal_time_constant=[.001, .2] s  thermal_time_constant_Cauer=[.001, .1, .2] s  thermal_time_constant_Foster=[7e-05, .0007, .01, .08] s  thermal_mass_initial_temperatures=[25, 25] degC  thermal_mass_initial_temperatures_Cauer=[25, 25, 25] degC  junction_thermal_mass=0.01 J/K  steadyState_Foster=simscape.enum.onoff.on  Tvec_initial_Foster=[25, 25, 25, 25] degC  no_thermal_network=0  junction_temperature_specify=off  junction_temperature_priority=None  junction_temperature=25 degC  junction_temperature_nominal_specify=off  junction_temperature_nominal_unit=degC  junction_temperature_nominal_value=1  vT_specify=off  vT_priority=None  vT=0 V  vT_nominal_specify=off  vT_nominal_unit=V  vT_nominal_value=1  Qj_specify=off  Qj_priority=None  Qj=0 W  Qj_nominal_specify=off  Qj_nominal_unit=W  Qj_nominal_value=1
  IGBT C(H) : ee_lib/Semiconductors & Converters/IGBT (Ideal, Switching)  Vf=0.8 V  Ron=0.001 Ohm  Goff=1e-5 S  Vth=0.5 V  diode_param=2  diode_Vf=0.8 V  diode_Ron=0.001 Ohm  diode_Goff=1e-5 S  diode_C=5e-8 F  diode_iRM=-235 A  diode_iF=300 A  diode_idot=-50 A/us  diode_trr_param=1  diode_trr_factor=3  diode_trr=15 us  diode_Qrr=1.5e+3 s*uA  thermal_loss_option=ee.enum.converters.thermalLossOption.constantvalues  Von_data=[0, .1, .6, .8, 1, 1.3, 1.6, 2, 2.4; 0, .1, .7, 1, 1.2, 1.5, 1.9, 2.4, 2.8] V  Tj=[298.15, 398.15] K  Iout_data=[0, .1, 1, 5, 10, 20, 40, 70, 100] A  Eon_data=[0, .0024, .024, .12, .2, .48, 1.04, 2.16, 3.24; 0, .003, .03, .15, .25, .6, 1.3, 2.7, 4.05] * 1e-3 J  Eoff_data=[0, .0007, .0066, .033, .066, .17, .33, .83, 1.5; 0, .001, .01, .05, .1, .25, .5, 1.2, 2.2] * 1e-3 J  Tj_loss=[298.15, 398.15] K  Iout_data_loss=[0, .1, 1, 5, 10, 20, 40, 70, 100] A  Eon_scalar=22.86e-3 J  Eoff_scalar=17.14e-3 J  Voff=300 V  Iout_scalar=600 A  diodeModelType=ee.enum.converters.diodeModelType.pwl  diodeTableType=ee.enum.diode.tableType.IfMat  diode_IfMat=[.07, .12, .19, 1.75, 4.24, 7.32, 11.2; .16, .3, .72, 2.14, 4.02, 6.35, 9.12] A  diode_VfMat=[.9, 1.15, 1.25, 1.5, 1.75, 2.17, 2.6, 2.85; .58, .68, .75, 1.1, 1.38, 1.77, 2.27, 2.7] V  diode_TjVec=[25, 125] degC  diode_VfVec=[.5, .7, .9, 1.3, 1.7, 2.1, 2.5] V  diode_IfVec=[.1, .2, .5, 1, 2, 4, 7, 10] A  diode_Vr=-600 V  diode_Ls=150 nH  diode_Erec=0.03 J  thermal_network_parameterization=ee.enum.thermalNetworkTopology.external  Rth=[.08, .5] K/W  Rth_Cauer=[.08, .1, .5] K/W  Rth_Foster=[.08, .14, .22, .16] K/W  thermal_mass_parameterization=ee.enum.thermalNetwork.timeconstant  thermal_mass=[.01, .5] J/K  thermal_mass_Cauer=[.01, .1, .5] J/K  thermal_mass_Foster=[.001, .005, .05, .5] J/K  thermal_time_constant=[.001, .2] s  thermal_time_constant_Cauer=[.001, .1, .2] s  thermal_time_constant_Foster=[7e-05, .0007, .01, .08] s  thermal_mass_initial_temperatures=[25, 25] degC  thermal_mass_initial_temperatures_Cauer=[25, 25, 25] degC  junction_thermal_mass=0.01 J/K  steadyState_Foster=simscape.enum.onoff.on  Tvec_initial_Foster=[25, 25, 25, 25] degC  no_thermal_network=0  junction_temperature_specify=off  junction_temperature_priority=None  junction_temperature=25 degC  junction_temperature_nominal_specify=off  junction_temperature_nominal_unit=degC  junction_temperature_nominal_value=1  vT_specify=off  vT_priority=None  vT=0 V  vT_nominal_specify=off  vT_nominal_unit=V  vT_nominal_value=1  Qj_specify=off  Qj_priority=None  Qj=0 W  Qj_nominal_specify=off  Qj_nominal_unit=W  Qj_nominal_value=1
  IGBT C(L) : ee_lib/Semiconductors & Converters/IGBT (Ideal, Switching)  Vf=0.8 V  Ron=0.001 Ohm  Goff=1e-5 S  Vth=0.5 V  diode_param=2  diode_Vf=0.8 V  diode_Ron=0.001 Ohm  diode_Goff=1e-5 S  diode_C=5e-8 F  diode_iRM=-235 A  diode_iF=300 A  diode_idot=-50 A/us  diode_trr_param=1  diode_trr_factor=3  diode_trr=15 us  diode_Qrr=1.5e+3 s*uA  thermal_loss_option=ee.enum.converters.thermalLossOption.constantvalues  Von_data=[0, .1, .6, .8, 1, 1.3, 1.6, 2, 2.4; 0, .1, .7, 1, 1.2, 1.5, 1.9, 2.4, 2.8] V  Tj=[298.15, 398.15] K  Iout_data=[0, .1, 1, 5, 10, 20, 40, 70, 100] A  Eon_data=[0, .0024, .024, .12, .2, .48, 1.04, 2.16, 3.24; 0, .003, .03, .15, .25, .6, 1.3, 2.7, 4.05] * 1e-3 J  Eoff_data=[0, .0007, .0066, .033, .066, .17, .33, .83, 1.5; 0, .001, .01, .05, .1, .25, .5, 1.2, 2.2] * 1e-3 J  Tj_loss=[298.15, 398.15] K  Iout_data_loss=[0, .1, 1, 5, 10, 20, 40, 70, 100] A  Eon_scalar=22.86e-3 J  Eoff_scalar=17.14e-3 J  Voff=300 V  Iout_scalar=600 A  diodeModelType=ee.enum.converters.diodeModelType.pwl  diodeTableType=ee.enum.diode.tableType.IfMat  diode_IfMat=[.07, .12, .19, 1.75, 4.24, 7.32, 11.2; .16, .3, .72, 2.14, 4.02, 6.35, 9.12] A  diode_VfMat=[.9, 1.15, 1.25, 1.5, 1.75, 2.17, 2.6, 2.85; .58, .68, .75, 1.1, 1.38, 1.77, 2.27, 2.7] V  diode_TjVec=[25, 125] degC  diode_VfVec=[.5, .7, .9, 1.3, 1.7, 2.1, 2.5] V  diode_IfVec=[.1, .2, .5, 1, 2, 4, 7, 10] A  diode_Vr=-600 V  diode_Ls=150 nH  diode_Erec=0.03 J  thermal_network_parameterization=ee.enum.thermalNetworkTopology.external  Rth=[.08, .5] K/W  Rth_Cauer=[.08, .1, .5] K/W  Rth_Foster=[.08, .14, .22, .16] K/W  thermal_mass_parameterization=ee.enum.thermalNetwork.timeconstant  thermal_mass=[.01, .5] J/K  thermal_mass_Cauer=[.01, .1, .5] J/K  thermal_mass_Foster=[.001, .005, .05, .5] J/K  thermal_time_constant=[.001, .2] s  thermal_time_constant_Cauer=[.001, .1, .2] s  thermal_time_constant_Foster=[7e-05, .0007, .01, .08] s  thermal_mass_initial_temperatures=[25, 25] degC  thermal_mass_initial_temperatures_Cauer=[25, 25, 25] degC  junction_thermal_mass=0.01 J/K  steadyState_Foster=simscape.enum.onoff.on  Tvec_initial_Foster=[25, 25, 25, 25] degC  no_thermal_network=0  junction_temperature_specify=off  junction_temperature_priority=None  junction_temperature=25 degC  junction_temperature_nominal_specify=off  junction_temperature_nominal_unit=degC  junction_temperature_nominal_value=1  vT_specify=off  vT_priority=None  vT=0 V  vT_nominal_specify=off  vT_nominal_unit=V  vT_nominal_value=1  Qj_specify=off  Qj_priority=None  Qj=0 W  Qj_nominal_specify=off  Qj_nominal_unit=W  Qj_nominal_value=1
  Phase Splitter : ee_lib/Connectors & References/Phase Splitter
      settings: SourceProductBaseCode=PS
  Simulink-PS G{1..6} (6 alike) : nesl_utility/Simulink-PS Converter  PhysicalDomain=network_engine_domain  SubClassName=ps_input  LeftPortType=input  RightPortType=output  PseudoPeriodic=off  Frequencies=[]  NoiseDistribution=none  NoiseParameters=[]  Unit=1  AffineConversion=off  FilteringAndDerivatives=zero  SimscapeFilterOrder=1  InputFilterTimeConstant=1e-6  UdotUserProvided=0
      settings: SourceProductBaseCode=SS,PW,VE
  24V+ : PMIOPort  Side=Left
  0 : PMIOPort  Port=2  Side=Left
  iabc : PMIOPort  Port=3  Side=Right
  wires:
  Demux/1 -> Simulink-PS G1/1
  Demux/3 -> Simulink-PS G3/1
  Demux/2 -> Simulink-PS G2/1
  Demux/4 -> Simulink-PS G4/1
  Demux/5 -> Simulink-PS G5/1
  Demux/6 -> Simulink-PS G6/1
  G/1 -> Demux/1
  connections:
  IGBT C(H)/RConn1 -- IGBT B(H)/RConn1 -- 24V+/RConn1 -- IGBT A(H)/RConn1
  IGBT C(L)/RConn2 -- IGBT B(L)/RConn2 -- 0/RConn1 -- IGBT A(L)/RConn2
  IGBT C(L)/RConn1 -- IGBT C(H)/RConn2 -- Phase Splitter/RConn3
  IGBT A(L)/LConn1 -- Simulink-PS G2/RConn1
  IGBT B(L)/LConn1 -- Simulink-PS G4/RConn1
  Simulink-PS G1/RConn1 -- IGBT A(H)/LConn1
  IGBT B(L)/RConn1 -- IGBT B(H)/RConn2 -- Phase Splitter/RConn2
  IGBT A(H)/RConn2 -- IGBT A(L)/RConn1 -- Phase Splitter/RConn1
  iabc/RConn1 -- Phase Splitter/LConn1
  IGBT C(L)/LConn1 -- Simulink-PS G6/RConn1
  IGBT B(H)/LConn1 -- Simulink-PS G3/RConn1
  IGBT C(H)/LConn1 -- Simulink-PS G5/RConn1
